simulink model "td1_4"  (R2023a)
settings: Solver=VariableStepAuto  StartTime=0.0  StopTime=10.0  RelTol=1e-3
libraries: mpclib x1, cstblocks x1
settings Model: Creator=z92504194  LastModifiedBy=z92504194

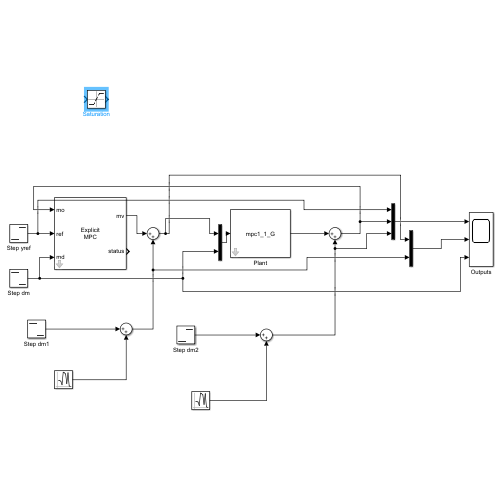
[thumbnail: Simulink's stored preview of the top-level diagram]
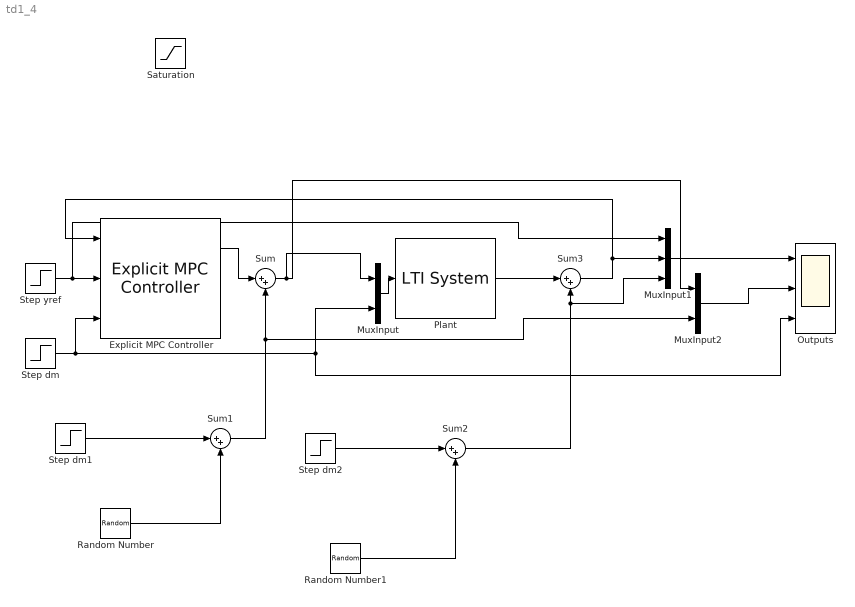
== system td1_4 ==
  Explicit MPC Controller : mpclib/Explicit MPC Controller  SCDEnableBlockLinearizationSpecification=on  empcobj=mpc1E  is_multiple=0  enable_value=0  return_u0=off  md_inport=on  mv_inport=off  return_status=on  return_region=off  return_state=off  state_inport=off  BlockDataType=double  SampleTimeInherited=off  switch_inport=off
  MuxInput : Mux  Inputs=2
  MuxInput1 : Mux  Inputs=3
  MuxInput2 : Mux  Inputs=2
  Outputs : Scope  NumInputPorts=3
  Plant : cstblocks/LTI System  sys=mpc1_1_G  IC=[]
  Random Number : RandomNumber  Variance=0.0001  SampleTime=0.5
  Random Number1 : RandomNumber  Variance=0.0001  SampleTime=0.5
  Saturation : Saturate
  Step dm : Step  Time=20  After=-5
  Step dm1 : Step  Time=50  After=-0.1
  Step dm2 : Step  Time=30
  Step yref : Step  Time=10  After=20
  Sum{,1..3} (4 alike) : Sum  Inputs=|++
  wires:
  Step yref/1 -> Explicit MPC Controller/2, MuxInput1/1
  Step dm/1 -> Explicit MPC Controller/3, MuxInput/2, Outputs/3
  MuxInput/1 -> Plant/1
  Step dm2/1 -> Sum2/1
  Sum1/1 -> MuxInput2/2, Sum/2
  Plant/1 -> Sum3/1
  Random Number/1 -> Sum1/2
  MuxInput1/1 -> Outputs/1
  Step dm1/1 -> Sum1/1
  Random Number1/1 -> Sum2/2
  MuxInput2/1 -> Outputs/2
  Sum3/1 -> Explicit MPC Controller/1, MuxInput1/2
  Explicit MPC Controller/1 -> Sum/1
  Sum/1 -> MuxInput/1, MuxInput2/1
  Sum2/1 -> MuxInput1/3, Sum3/2
